simulink model "SIXDOF28"  (R2025b)
settings: Solver=VariableStepAuto  StartTime=0.0  StopTime=sortieStopTime_s  MaxStep=2.0  RelTol=1e-3
undefined symbols (not defined in the file): aircraft_mass, alpha0, alpha_bp, b, CL_table, ClCsurfaces, Cldampingrates, Cldeltae, CmCsurfaces, Cmdampingrates, CnCsurfaces, Cndampingrates, COP, CruiseSpeed, deg, density, DiscIntNeverNeededParam, dwGrad, ElTrim, g, h0, InitialHeadingRadBySortie, InitialPosBySortie, InitPitch, InitUb, Initwb, l, lt, maxPropRad, payloadvolume, PitchTrim, rad, rho, s, S, selectedSortie, St, ThrottleTrim
libraries: slpidlib x12, aerolibasang x3, aerolibconvert2 x2, aerolibadyn x1
(part 1 of 3)
settings Model: Creator=User  LastModifiedBy=User
settings SolverCC: ZeroCrossAlgorithm=Adaptive
settings DataIOCC: ExternalInput=getinputstruct(SIXDOF17TRIM)  InitialState=getstatestruct(SIXDOF17TRIM)  Refine=5
settings DebuggingCC: MaskedZcDiagnostic=none  IgnoredZcDiagnostic=none

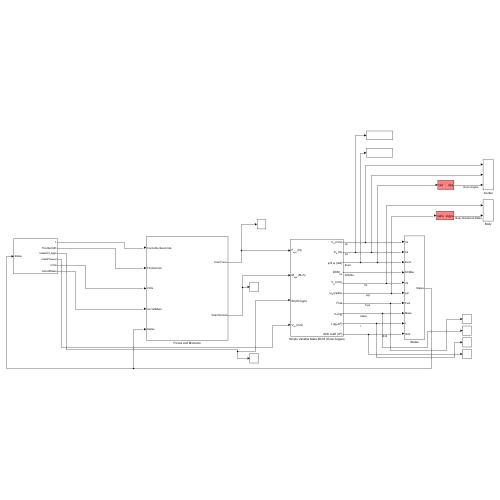
[thumbnail: Simulink's stored preview of the top-level diagram]
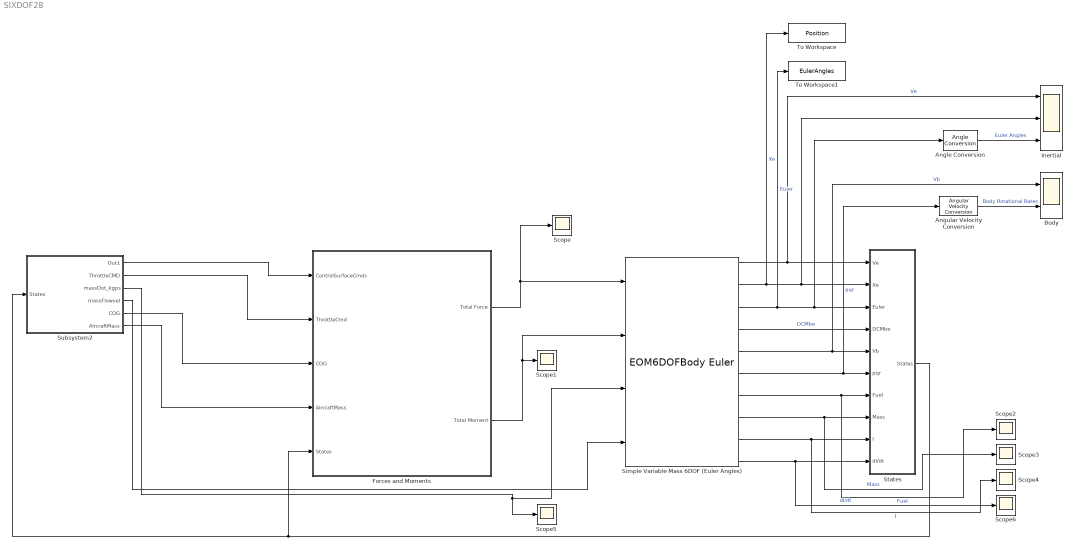
== system SIXDOF28 ==
  Angle Conversion : aerolibconvert2/Angle Conversion  IU=rad  OU=deg
  Angular Velocity Conversion : aerolibconvert2/Angular Velocity Conversion  IU=rad/s  OU=deg/s
  Body : Scope  NumInputPorts=2
      settings: TimeSpan=10  ActiveDisplayYMinimum=-7.1173373143171261  ActiveDisplayYMaximum=39.342522904173691
  Forces and Moments : Subsystem
  Inertial : Scope  NumInputPorts=3
      settings: TimeSpan=10  ActiveDisplayYMinimum=-30.17741938857975  ActiveDisplayYMaximum=31.493242322208388  DataLoggingVariableName=InertialData
  Scope{,1..6} (7 alike) : Scope
      Scope settings: ActiveDisplayYMinimum=-1086.3345140909432  ActiveDisplayYMaximum=956.25135632506715  DataLoggingVariableName=ScopeData65
      Scope1 settings: ActiveDisplayYMinimum=-0.001966592183015876  ActiveDisplayYMaximum=0.0097082532484662285  DataLoggingVariableName=ScopeData66
      Scope2 settings: ActiveDisplayYMinimum=-1  ActiveDisplayYMaximum=1  DataLoggingVariableName=ScopeData57
      Scope3 settings: ActiveDisplayYMinimum=92.2325499999995  ActiveDisplayYMaximum=150.86305000000004  DataLoggingVariableName=ScopeData60
      Scope4 settings: DataLoggingVariableName=ScopeData82
      Scope5 settings: ActiveDisplayYMinimum=-1  ActiveDisplayYMaximum=1  DataLoggingVariableName=ScopeData120
      Scope6 settings: DataLoggingVariableName=ScopeData92
  Simple Variable Mass 6DOF (Euler Angles) : EOM6DOFBodyEuler  mtype=Simple Variable  xme_0=InitialPosBySortie(selectedSortie,:)  Vm_0=[InitUb 0 Initwb]  eul_0=[0 InitPitch InitialHeadingRadBySortie(selectedSortie)]  mass_0=aircraft_mass  mass_e=emptymass  mass_f=aircraft_mass  inertia_e=EmptyInertiaMatrix  inertia_f=FullInertiaMatrix  vre_flag=on  mass_flag=on
  States : Subsystem
  Subsystem2 : Subsystem
  To Workspace : ToWorkspace  VariableName=Position  SaveFormat=Timeseries  SampleTime=-1
  To Workspace1 : ToWorkspace  VariableName=EulerAngles  SaveFormat=Timeseries  SampleTime=-1
  wires:
  Angle Conversion/1 -> Inertial/3  "Euler Angles"
  Angular Velocity Conversion/1 -> Body/2  "Body Rotational Rates"
  States/1(States) -> Subsystem2/1(States), Forces and Moments/5(States)
  Subsystem2/1(Out1) -> Forces and Moments/1(ControlSurfaceCmds)
  Forces and Moments/1(Total Force) -> Simple Variable Mass 6DOF (Euler Angles)/1, Scope/1
  Forces and Moments/2(Total Moment) -> Simple Variable Mass 6DOF (Euler Angles)/2, Scope1/1
  Subsystem2/2(ThrottleCMD) -> Forces and Moments/2(ThrottleCmd)
  Subsystem2/3(massDot_kgps) -> Simple Variable Mass 6DOF (Euler Angles)/3, Scope5/1
  Subsystem2/4(massFlowvel) -> Simple Variable Mass 6DOF (Euler Angles)/4
  Subsystem2/5(COG) -> Forces and Moments/3(COG)
  Subsystem2/6(AircraftMass) -> Forces and Moments/4(AircraftMass)
  Simple Variable Mass 6DOF (Euler Angles)/1 -> States/1(Ve), Inertial/1  "Ve"
  Simple Variable Mass 6DOF (Euler Angles)/2 -> To Workspace/1, States/2(Xe), Inertial/2  "Xe"
  Simple Variable Mass 6DOF (Euler Angles)/3 -> To Workspace1/1, States/3(Euler), Angle Conversion/1  "Euler"
  Simple Variable Mass 6DOF (Euler Angles)/4 -> States/4(DCMbe)  "DCMbe"
  Simple Variable Mass 6DOF (Euler Angles)/5 -> Body/1, States/5(Vb)  "Vb"
  Simple Variable Mass 6DOF (Euler Angles)/6 -> Angular Velocity Conversion/1, States/6(pqr)  "pqr"
  Simple Variable Mass 6DOF (Euler Angles)/7 -> Scope2/1, States/7(Fuel)  "Fuel"
  Simple Variable Mass 6DOF (Euler Angles)/8 -> Scope3/1, States/8(Mass)  "Mass"
  Simple Variable Mass 6DOF (Euler Angles)/9 -> Scope4/1, States/9(I)  "I"
  Simple Variable Mass 6DOF (Euler Angles)/10 -> Scope6/1, States/10(dI/dt)  "dI/dt"

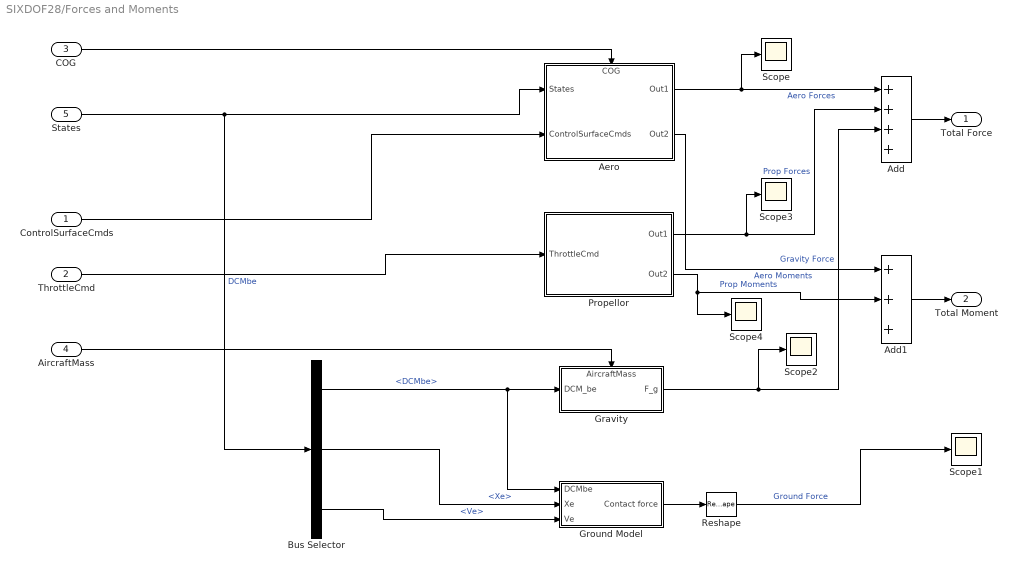
== system SIXDOF28/Forces and Moments ==
  ControlSurfaceCmds : Inport
  ThrottleCmd : Inport  Port=2
  COG : Inport  Port=3
  AircraftMass : Inport  Port=4
  States : Inport  Port=5
  Add : Sum  Inputs=++++
  Add1 : Sum  Inputs=+++
  Aero : Subsystem
      settings: PortSchema="{\"entries\":[{\"content\":{\"sides\":[{\"content\":{\"connectorIds\":[\"In1\",\"In2\"]},\"type\":\"ConnectorPlacement.EquallySpacedRectSide\",\"uuid\":\"609f64a6-fe2d-463f-8571-6107a2609829\"},{\"content\":{\"connectorIds\":[\"Out1\",\"Out2\"],\"side\":\"RIGHT\"},\"type\":\"ConnectorPlacement.EquallySpacedRectSide\",\"uuid\":\"636f2898-b73d-43f5-aead-2dc1a8211e6d\"},{\"content\":{\"connectorIds\":[\"In3\"],\"side\":\"TOP\"},\"type\":\"ConnectorPlacement.EquallySpacedRectSide\",\"uuid\":\"2beb2726-5e66-44a5-8496-281bf40e3bd0\"}]},\"type\":\"ConnectorPlacement.EquallySpacedConnector\",\"uuid\":\"f99eef0b-ac9c-4788-9a1a-1fc150c0b76e\"}],\"packageUris\":[\"http://schema.mathworks.com/mf0/Connector/R2020b\"],\"version\":\"1.0\"}"
  Bus Selector : BusSelector  OutputSignals=DCMbe,Xe,Ve
  Gravity : Subsystem
      settings: PortSchema="{\"entries\":[{\"content\":{\"sides\":[{\"content\":{\"connectorIds\":[\"In1\"]},\"type\":\"ConnectorPlacement.EquallySpacedRectSide\",\"uuid\":\"63d9ec0b-6663-4eeb-9ffd-c4a1f3d6fae8\"},{\"content\":{\"connectorIds\":[\"Out1\"],\"side\":\"RIGHT\"},\"type\":\"ConnectorPlacement.EquallySpacedRectSide\",\"uuid\":\"9033ce56-a827-4af9-9d8f-92169c025264\"},{\"content\":{\"connectorIds\":[\"In2\"],\"side\":\"TOP\"},\"type\":\"ConnectorPlacement.EquallySpacedRectSide\",\"uuid\":\"84568abc-cdbf-45a7-a6af-9a5fdbdb6515\"}]},\"type\":\"ConnectorPlacement.EquallySpacedConnector\",\"uuid\":\"857b6717-75e8-42d2-8d9f-18d4eadb3b26\"}],\"packageUris\":[\"http://schema.mathworks.com/mf0/Connector/R2020b\"],\"version\":\"1.0\"}"
  Ground Model : Subsystem
  Propellor : Subsystem
  Reshape : Reshape
  Scope{,1..4} (5 alike) : Scope
      Scope settings: ActiveDisplayYMinimum=-2618.1799390430056  ActiveDisplayYMaximum=542.63664124652109  DataLoggingVariableName=ScopeData40
      Scope1 settings: ActiveDisplayYMinimum=-1  ActiveDisplayYMaximum=1  DataLoggingVariableName=ScopeData43
      Scope2 settings: ActiveDisplayYMinimum=-236.10201419942058  ActiveDisplayYMaximum=1116.233557133269  DataLoggingVariableName=ScopeData44
      Scope3 settings: ActiveDisplayYMinimum=-38.137986036605241  ActiveDisplayYMaximum=343.24187432944723  DataLoggingVariableName=ScopeData54
      Scope4 settings: ActiveDisplayYMinimum=-19.196026162968661  ActiveDisplayYMaximum=172.764235466718  DataLoggingVariableName=ScopeData80
  Total Force : Outport
  Total Moment : Outport  Port=2
  wires:
  Add/1 -> Total Force/1
  Add1/1 -> Total Moment/1
  States/1 -> Bus Selector/1, Aero/1(States)  "DCMbe"
  Bus Selector/1 -> Ground Model/1(DCMbe), Gravity/1(DCM_be)  "<DCMbe>"
  Bus Selector/2 -> Ground Model/2(Xe)  "<Xe>"
  Bus Selector/3 -> Ground Model/3(Ve)  "<Ve>"
  Ground Model/1(Contact force) -> Reshape/1
  Reshape/1 -> Scope1/1  "Ground Force"
  Aero/1(Out1) -> Add/1, Scope/1  "Aero Forces"
  Gravity/1(F_g) -> Scope2/1, Add/3  "Gravity Force"
  ControlSurfaceCmds/1 -> Aero/2(ControlSurfaceCmds)
  Propellor/1(Out1) -> Scope3/1, Add/2  "Prop Forces"
  ThrottleCmd/1 -> Propellor/1(ThrottleCmd)
  Propellor/2(Out2) -> Add1/2, Scope4/1  "Prop Moments"
  Aero/2(Out2) -> Add1/1  "Aero Moments"
  COG/1 -> Aero/3(COG)
  AircraftMass/1 -> Gravity/2(AircraftMass)

== system SIXDOF28/States ==
  Ve : Inport
  Xe : Inport  Port=2
  Euler : Inport  Port=3
  DCMbe : Inport  Port=4
  Vb : Inport  Port=5
  pqr : Inport  Port=6
  Fuel : Inport  Port=7
  Mass : Inport  Port=8
  I : Inport  Port=9
  dI/dt : Inport  Port=10
  Atan2 : Trigonometry  Operator=atan2
  Bus Creator : BusCreator  Inputs=11
  Selector : Selector  InputPortWidth=3  IndexOptions=Index vector (dialog)  Indices=[2]  OutputSizes=1
  Selector1 : Selector  InputPortWidth=3  IndexOptions=Index vector (dialog)  Indices=[1]  OutputSizes=1
  States : Outport
  wires:
  Bus Creator/1 -> States/1
  Ve/1 -> Selector1/1, Selector/1, Bus Creator/1
  Xe/1 -> Bus Creator/2
  Euler/1 -> Bus Creator/3
  DCMbe/1 -> Bus Creator/4
  Vb/1 -> Bus Creator/5
  pqr/1 -> Bus Creator/6
  Fuel/1 -> Bus Creator/7
  Mass/1 -> Bus Creator/8
  I/1 -> Bus Creator/9
  Selector/1 -> Atan2/1
  Selector1/1 -> Atan2/2
  Atan2/1 -> Bus Creator/11  "Heading"
  dI/dt/1 -> Bus Creator/10

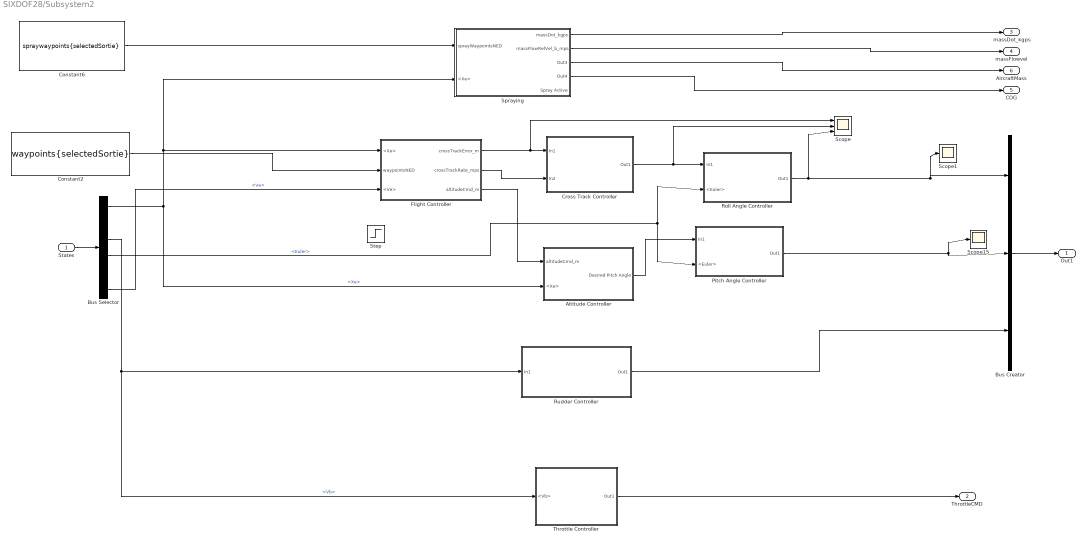
== system SIXDOF28/Subsystem2 ==
  States : Inport
  Altitude Controller : Subsystem
  Bus Creator : BusCreator  Inputs=3
  Bus Selector : BusSelector  OutputSignals=Xe,pqr,Vb,Euler,Heading,Ve
  Constant2 : Constant  Value=waypoints{selectedSortie}
  Constant6 : Constant  Value=spraywaypoints{selectedSortie}
  Cross Track Controller : Subsystem
  Flight Controller : Subsystem
  Pitch Angle Controller : Subsystem
  Roll Angle Controller : Subsystem
  Rudder Controller : Subsystem
  Scope : Scope  NumInputPorts=3
      settings: ActiveDisplayYMinimum=-1  ActiveDisplayYMaximum=1  DataLoggingVariableName=ScopeData85
  Scope1 : Scope
      settings: DataLoggingVariableName=ScopeData86
  Scope15 : Scope
      settings: ActiveDisplayYMinimum=-0.51269046777333427  ActiveDisplayYMaximum=0.25089107997418486  DataLoggingVariableName=ScopeData84
  Spraying : Subsystem
  Step : Step  Time=50  Before=4  After=20  SampleTime=0
  Throttle Controller : Subsystem
  Out1 : Outport
  ThrottleCMD : Outport  Port=2
  massDot_kgps : Outport  Port=3
  massFlowvel : Outport  Port=4
  COG : Outport  Port=5
  AircraftMass : Outport  Port=6
  wires:
  States/1 -> Bus Selector/1
  Bus Creator/1 -> Out1/1
  Altitude Controller/1(Desired Pitch Angle) -> Pitch Angle Controller/1(In1)
  Bus Selector/1 -> Altitude Controller/2(<Xe>), Spraying/2(<Xe>), Flight Controller/1(<Xe>)  "<Xe>"
  Pitch Angle Controller/1(Out1) -> Bus Creator/2, Scope15/1
  Bus Selector/4 -> Pitch Angle Controller/2(<Euler>), Roll Angle Controller/2(<Euler>)  "<Euler>"
  Roll Angle Controller/1(Out1) -> Scope/3, Bus Creator/1, Scope1/1
  Bus Selector/3 -> Rudder Controller/1(In1), Throttle Controller/1(<Vb>)  "<Vb>"
  Throttle Controller/1(Out1) -> ThrottleCMD/1
  Cross Track Controller/1(Out1) -> Scope/2, Roll Angle Controller/1(In1)
  Bus Selector/6 -> Flight Controller/3(<Ve>)  "<Ve>"
  Flight Controller/1(crossTrackError_m) -> Scope/1, Cross Track Controller/1(In1)
  Flight Controller/2(crossTrackRate_mps) -> Cross Track Controller/2(In2)
  Spraying/1(massDot_kgps) -> massDot_kgps/1
  Spraying/2(massFlowRelVel_b_mps) -> massFlowvel/1
  Spraying/3(Out3) -> AircraftMass/1
  Spraying/4(Out4) -> COG/1
  Flight Controller/3(altitudeCmd_m) -> Altitude Controller/1(altitudeCmd_m)
  Constant2/1 -> Flight Controller/2(waypointsNED)
  Constant6/1 -> Spraying/1(sprayWaypointsNED)
  Rudder Controller/1(Out1) -> Bus Creator/3

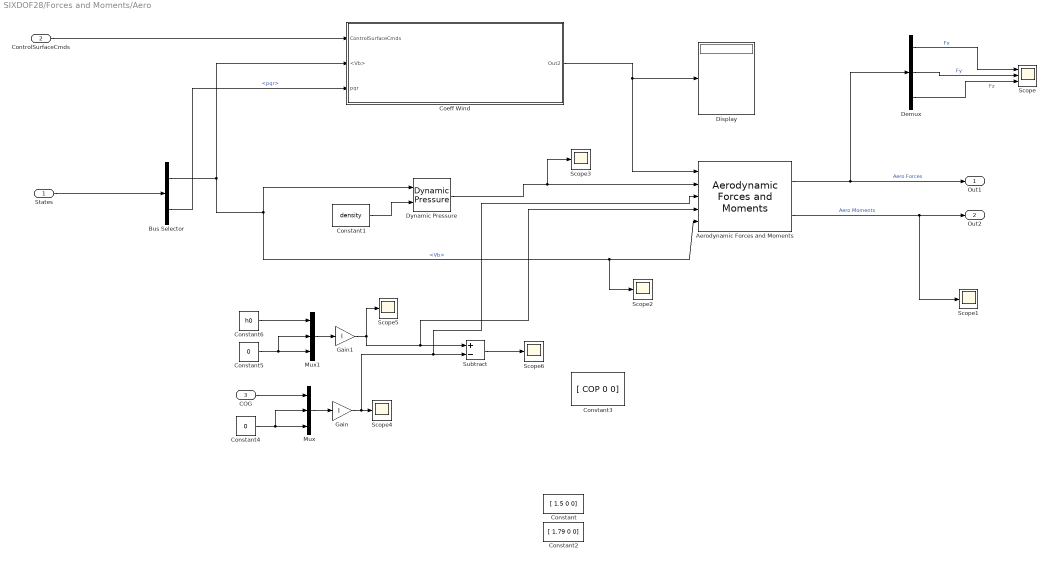
== system SIXDOF28/Forces and Moments/Aero ==
  States : Inport
  ControlSurfaceCmds : Inport  Port=2
  COG : Inport  Port=3
  "Aerodynamic Forces and Moments " : aerolibadyn/Aerodynamic Forces and Moments   inputAxes=Wind  outputForceAxes=Body  outputMomentAxes=Body  S=S  b=b  cbar=l
  Bus Selector : BusSelector  OutputSignals=Vb,pqr
  Coeff Wind : Subsystem
  Constant : Constant  Value=[ 1.5 0 0]
  Constant1 : Constant  Value=density
  Constant2 : Constant  Value=[ 1.79 0 0]
  Constant3 : Constant  Value=[ COP 0 0]
  Constant4 : Constant  Value=0
  Constant5 : Constant  Value=0
  Constant6 : Constant  Value=h0
  Demux : Demux  Outputs=3
  Display : Display
  Dynamic Pressure : aerolibasang/Dynamic Pressure
  Gain : Gain  Gain=l
  Gain1 : Gain  Gain=l
  Mux : Mux  Inputs=3
  Mux1 : Mux  Inputs=3
  Scope : Scope  NumInputPorts=3
      settings: ActiveDisplayYMinimum=-2654.35797194935  ActiveDisplayYMaximum=770.34591129163266  DataLoggingVariableName=ScopeData13
  Scope{1..6} (6 alike) : Scope
      Scope1 settings: ActiveDisplayYMinimum=-1  ActiveDisplayYMaximum=1  DataLoggingVariableName=ScopeData14
      Scope2 settings: ActiveDisplayYMinimum=-1  ActiveDisplayYMaximum=1
      Scope3 settings: ActiveDisplayYMinimum=-1  ActiveDisplayYMaximum=1  DataLoggingVariableName=ScopeData2
      Scope4 settings: ActiveDisplayYMinimum=-1  ActiveDisplayYMaximum=1  DataLoggingVariableName=ScopeData125
      Scope5 settings: ActiveDisplayYMinimum=-1  ActiveDisplayYMaximum=1  DataLoggingVariableName=ScopeData126
      Scope6 settings: ActiveDisplayYMinimum=-1  ActiveDisplayYMaximum=1  DataLoggingVariableName=ScopeData127
  Subtract : Sum  Inputs=+-
  Out1 : Outport
  Out2 : Outport  Port=2
  wires:
  "Aerodynamic Forces and Moments "/1 -> Demux/1, Out1/1  "Aero Forces"
  "Aerodynamic Forces and Moments "/2 -> Scope1/1, Out2/1  "Aero Moments"
  Constant1/1 -> Dynamic Pressure/2
  Dynamic Pressure/1 -> Scope3/1, "Aerodynamic Forces and Moments "/2
  States/1 -> Bus Selector/1
  Bus Selector/1 -> Scope2/1, "Aerodynamic Forces and Moments "/5, Dynamic Pressure/1, Coeff Wind/2(<Vb>)  "<Vb>"
  Coeff Wind/1(Out2) -> "Aerodynamic Forces and Moments "/1, Display/1
  Demux/2 -> Scope/2  "Fy"
  Demux/1 -> Scope/1  "Fx"
  Demux/3 -> Scope/3  "Fz"
  Bus Selector/2 -> Coeff Wind/3(pqr)  "<pqr>"
  ControlSurfaceCmds/1 -> Coeff Wind/1(ControlSurfaceCmds)
  COG/1 -> Mux/1
  Constant4/1 -> Mux/2, Mux/3
  Mux/1 -> Gain/1
  Gain/1 -> "Aerodynamic Forces and Moments "/3, Subtract/2, Scope4/1
  Constant5/1 -> Mux1/2, Mux1/3
  Constant6/1 -> Mux1/1
  Mux1/1 -> Gain1/1
  Gain1/1 -> Scope5/1, "Aerodynamic Forces and Moments "/4, Subtract/1
  Subtract/1 -> Scope6/1

== system SIXDOF28/Forces and Moments/Gravity ==
  DCM_be : Inport
  AircraftMass : Inport  Port=2
  Constant : Constant  Value=[ 0 0 g]
  MatrixMultiply : Product  Multiplication=Matrix(*)
  Product : Product
  F_g : Outport
  wires:
  Constant/1 -> MatrixMultiply/2
  DCM_be/1 -> MatrixMultiply/1
  MatrixMultiply/1 -> Product/2
  Product/1 -> F_g/1
  AircraftMass/1 -> Product/1

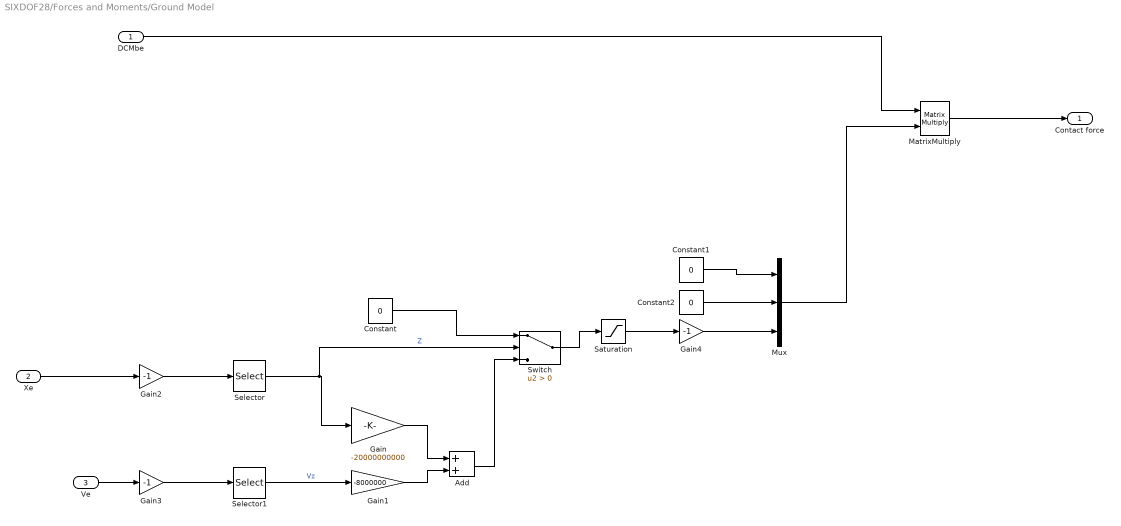
== system SIXDOF28/Forces and Moments/Ground Model ==
  DCMbe : Inport
  Xe : Inport  Port=2
  Ve : Inport  Port=3
  Add : Sum
  Constant : Constant  Value=0
  Constant1 : Constant  Value=0
  Constant2 : Constant  Value=0
  Gain : Gain  Gain=-20000000000
  Gain1 : Gain  Gain=-8000000
  Gain2 : Gain  Gain=-1
  Gain3 : Gain  Gain=-1
  Gain4 : Gain  Gain=-1
  MatrixMultiply : Product  Multiplication=Matrix(*)
  Mux : Mux  Inputs=3
  Saturation : Saturate  UpperLimit=inf  LowerLimit=-0.0
  Selector : Selector  InputPortWidth=3  IndexOptions=Index vector (dialog)  Indices=[3]  OutputSizes=1
  Selector1 : Selector  InputPortWidth=3  IndexOptions=Index vector (dialog)  Indices=[3]  OutputSizes=1
  Switch : Switch  Criteria=u2 > Threshold  SaturateOnIntegerOverflow=off  InputSameDT=off
  Contact force : Outport
  wires:
  Xe/1 -> Gain2/1
  Ve/1 -> Gain3/1
  Constant/1 -> Switch/1
  Gain/1 -> Add/1
  Gain1/1 -> Add/2
  Selector1/1 -> Gain1/1  "Vz"
  Selector/1 -> Switch/2, Gain/1  "Z"
  Add/1 -> Switch/3
  Gain2/1 -> Selector/1
  Gain3/1 -> Selector1/1
  Switch/1 -> Saturation/1
  DCMbe/1 -> MatrixMultiply/1
  MatrixMultiply/1 -> Contact force/1
  Gain4/1 -> Mux/3
  Constant2/1 -> Mux/2
  Constant1/1 -> Mux/1
  Saturation/1 -> Gain4/1
  Mux/1 -> MatrixMultiply/2

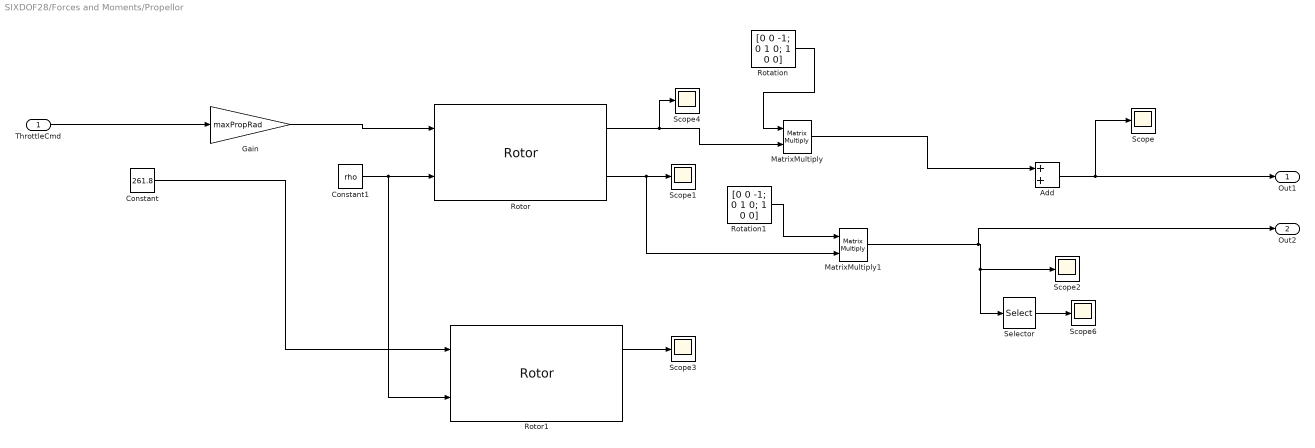
== system SIXDOF28/Forces and Moments/Propellor ==
  ThrottleCmd : Inport
  Add : Sum
  Constant : Constant  Value=261.8
  Constant1 : Constant  Value=rho
  Gain : Gain  Gain=maxPropRad
  MatrixMultiply : Product  Multiplication=Matrix(*)
  MatrixMultiply1 : Product  Multiplication=Matrix(*)
  Rotation : Constant  Value=[0 0 -1; 0 1 0; 1 0 0]
  Rotation1 : Constant  Value=[0 0 -1; 0 1 0; 1 0 0]
  Rotor : Rotor  CT=CT  CQ=CQ  radius=PropRadius
  Rotor1 : Rotor  radius=PropRadius
  Scope{,1..4,6} (6 alike) : Scope
      Scope settings: ActiveDisplayYMinimum=-1  ActiveDisplayYMaximum=1  DataLoggingVariableName=ScopeData18
      Scope1 settings: ActiveDisplayYMinimum=-1  ActiveDisplayYMaximum=1  DataLoggingVariableName=ScopeData19
      Scope2 settings: ActiveDisplayYMinimum=-0.90688934039232  ActiveDisplayYMaximum=8.1620040635308833  DataLoggingVariableName=ScopeData71
      Scope3 settings: ActiveDisplayYMinimum=-1  ActiveDisplayYMaximum=1  DataLoggingVariableName=ScopeData52
      Scope4 settings: ActiveDisplayYMinimum=-1  ActiveDisplayYMaximum=1  DataLoggingVariableName=ScopeData72
      Scope6 settings: ActiveDisplayYMinimum=-1  ActiveDisplayYMaximum=1  DataLoggingVariableName=ScopeData73
  Selector : Selector  InputPortWidth=3  IndexOptions=Index vector (dialog)  Indices=[ 1]  OutputSizes=1
  Out1 : Outport
  Out2 : Outport  Port=2
  wires:
  Constant1/1 -> Rotor1/2, Rotor/2
  Rotor/2 -> MatrixMultiply1/2, Scope1/1
  Add/1 -> Scope/1, Out1/1
  Rotor/1 -> Scope4/1, MatrixMultiply/2
  Rotation/1 -> MatrixMultiply/1
  MatrixMultiply/1 -> Add/1
  ThrottleCmd/1 -> Gain/1
  Rotation1/1 -> MatrixMultiply1/1
  MatrixMultiply1/1 -> Out2/1, Selector/1, Scope2/1
  Selector/1 -> Scope6/1
  Constant/1 -> Rotor1/1
  Rotor1/1 -> Scope3/1
  Gain/1 -> Rotor/1

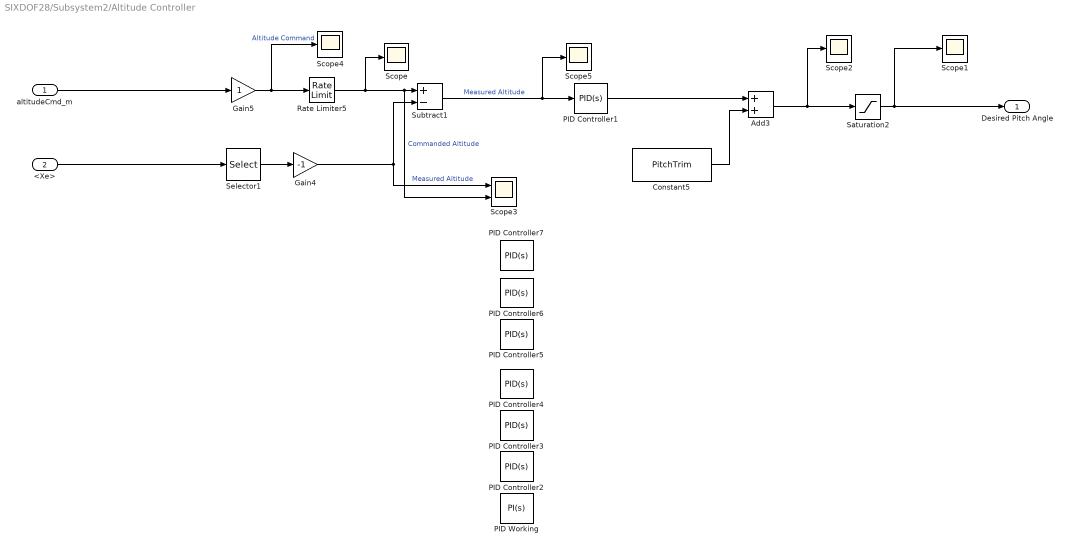
== system SIXDOF28/Subsystem2/Altitude Controller ==
  altitudeCmd_m : Inport
  <Xe> : Inport  Port=2
  Add3 : Sum
  Constant5 : Constant  Value=PitchTrim
  Gain4 : Gain  Gain=-1
  Gain5 : Gain
  PID Controller1 : slpidlib/PID Controller  Controller=PID  Form=Parallel  TimeDomain=Continuous-time  UseExternalTs=off  SampleTime=-1  IntegratorMethod=Forward Euler  FilterMethod=Forward Euler  ControllerParametersSource=internal  P=0.095  I=0.01  UseKiTs=off  D=0.07  UseExternalDerivativeSource=off  N=100  UseFilter=on  TunerSelectOption=Transfer Function Based (PID Tuner App)  InitialConditionSource=internal  InitialConditionForIntegrator=0  InitialConditionForFilter=0  DifferentiatorICPrevScaledInput=0  ExternalReset=none  TrackingMode=off  Kt=1  LimitOutput=off  SatLimitsSource=internal  UpperSaturationLimit=inf  LowerSaturationLimit=-inf  LinearizeAsGain=on  AntiWindupMode=none  Kb=1  LimitIntegrator=off  UpperIntegratorSaturationLimit=inf  LowerIntegratorSaturationLimit=-inf  POutMin=[]  POutMax=[]  IOutMin=[]  IOutMax=[]  DOutMin=[]  DOutMax=[]  NOutMin=[]  NOutMax=[]  SumOutMin=[]  SumOutMax=[]  SaturationOutMin=[]  SaturationOutMax=[]  PParamMin=[]  PParamMax=[]  IParamMin=[]  IParamMax=[]  DParamMin=[]  DParamMax=[]  NParamMin=[]  NParamMax=[]  KbParamMin=[]  KbParamMax=[]  KtParamMin=[]  KtParamMax=[]  KbOutMin=[]  KbOutMax=[]  KtOutMin=[]  KtOutMax=[]  IntegratorOutMin=[]  IntegratorOutMax=[]  FilterOutMin=[]  FilterOutMax=[]  SumI1OutMin=[]  SumI1OutMax=[]  SumI2OutMin=[]  SumI2OutMax=[]  SumI3OutMin=[]  SumI3OutMax=[]  SumI4OutMin=[]  SumI4OutMax=[]  SumDOutMin=[]  SumDOutMax=[]  DifferentiatorOutMin=[]  DifferentiatorOutMax=[]  FilterDiffOutCoefMin=[]  FilterDiffOutCoefMax=[]  ReciprocalOutMin=[]  ReciprocalOutMax=[]  SumDenOutMin=[]  SumDenOutMax=[]  SumNumOutMin=[]  SumNumOutMax=[]  DivideOutMin=[]  DivideOutMax=[]  UdiffTsProdOutMin=[]  UdiffTsProdOutMax=[]  NTsProdOutMin=[]  NTsProdOutMax=[]  UintegralTsProdOutMin=[]  UintegralTsProdOutMax=[]  UngainTsProdOutMin=[]  UngainTsProdOutMax=[]  ClampingZeroOutDataTypeStr=Inherit: Inherit via back propagation  ClampingZeroOutMin=[]  ClampingZeroOutMax=[]  FilterDenConstantOutDataTypeStr=Inherit: Inherit via back propagation  FilterDenConstantOutMin=[]  FilterDenConstantOutMax=[]  PCopyOutDataTypeStr=Inherit: Inherit via back propagation  PCopyOutMin=[]  PCopyOutMax=[]  NCopyOutDataTypeStr=Inherit: Inherit via back propagation  NCopyOutMin=[]  NCopyOutMax=[]  IntegratorContinuousStateAttributes=''  IntegratorStateMustResolveToSignalObject=off  IntegratorRTWStateStorageClass=Auto  FilterContinuousStateAttributes=''  FilterStateMustResolveToSignalObject=off  FilterRTWStateStorageClass=Auto  ParallelPVariant=InternalParameters  IdealPVariant=Disabled  IVariant=InternalParameters  DVariant=InternalParameters  IntegratorVariant=Continuous  SatVariant=Disabled  AWVariant=Passthrough  PCopyVariant=Disabled  TRVariant=Disabled  FdbkBlocksVariant=Forward  IdealPFdbkVariant=Disabled  SatFdbkVariant=Disabled  DerivativeFilterVariant=ContFilter  NVariant=InternalParameters  NCopyVariant=Disabled  FilterICVariant=InternalICsFilter  IntegratorICVariant=InternalICs  ExternalResetVariant=Disabled  TRSumVariant=Passthrough  SumFdbkVariant=Disabled  SumVariant=Sum_PID  TsampFilterVariant=InternalTs  TsampNgainVariant=Passthrough  TsampIntegralVariant=Disabled_SignalSpec  ExternalSaturationOutDataTypeStr=Inherit: Same as second input  DerivativeSourceVariant=ErrorSignal  PreIntVariant=InternalPreInt
  PID Controller2 : slpidlib/PID Controller  Controller=PID  Form=Parallel  TimeDomain=Continuous-time  UseExternalTs=off  SampleTime=-1  IntegratorMethod=Forward Euler  FilterMethod=Forward Euler  ControllerParametersSource=internal  P=0.1  I=0.01  UseKiTs=off  D=0.03  UseExternalDerivativeSource=off  N=100  UseFilter=on  TunerSelectOption=Transfer Function Based (PID Tuner App)  InitialConditionSource=internal  InitialConditionForIntegrator=0  InitialConditionForFilter=0  DifferentiatorICPrevScaledInput=0  ExternalReset=none  TrackingMode=off  Kt=1  LimitOutput=off  SatLimitsSource=internal  UpperSaturationLimit=inf  LowerSaturationLimit=-inf  LinearizeAsGain=on  AntiWindupMode=none  Kb=1  LimitIntegrator=off  UpperIntegratorSaturationLimit=inf  LowerIntegratorSaturationLimit=-inf  POutMin=[]  POutMax=[]  IOutMin=[]  IOutMax=[]  DOutMin=[]  DOutMax=[]  NOutMin=[]  NOutMax=[]  SumOutMin=[]  SumOutMax=[]  SaturationOutMin=[]  SaturationOutMax=[]  PParamMin=[]  PParamMax=[]  IParamMin=[]  IParamMax=[]  DParamMin=[]  DParamMax=[]  NParamMin=[]  NParamMax=[]  KbParamMin=[]  KbParamMax=[]  KtParamMin=[]  KtParamMax=[]  KbOutMin=[]  KbOutMax=[]  KtOutMin=[]  KtOutMax=[]  IntegratorOutMin=[]  IntegratorOutMax=[]  FilterOutMin=[]  FilterOutMax=[]  SumI1OutMin=[]  SumI1OutMax=[]  SumI2OutMin=[]  SumI2OutMax=[]  SumI3OutMin=[]  SumI3OutMax=[]  SumI4OutMin=[]  SumI4OutMax=[]  SumDOutMin=[]  SumDOutMax=[]  DifferentiatorOutMin=[]  DifferentiatorOutMax=[]  FilterDiffOutCoefMin=[]  FilterDiffOutCoefMax=[]  ReciprocalOutMin=[]  ReciprocalOutMax=[]  SumDenOutMin=[]  SumDenOutMax=[]  SumNumOutMin=[]  SumNumOutMax=[]  DivideOutMin=[]  DivideOutMax=[]  UdiffTsProdOutMin=[]  UdiffTsProdOutMax=[]  NTsProdOutMin=[]  NTsProdOutMax=[]  UintegralTsProdOutMin=[]  UintegralTsProdOutMax=[]  UngainTsProdOutMin=[]  UngainTsProdOutMax=[]  ClampingZeroOutDataTypeStr=Inherit: Inherit via back propagation  ClampingZeroOutMin=[]  ClampingZeroOutMax=[]  FilterDenConstantOutDataTypeStr=Inherit: Inherit via back propagation  FilterDenConstantOutMin=[]  FilterDenConstantOutMax=[]  PCopyOutDataTypeStr=Inherit: Inherit via back propagation  PCopyOutMin=[]  PCopyOutMax=[]  NCopyOutDataTypeStr=Inherit: Inherit via back propagation  NCopyOutMin=[]  NCopyOutMax=[]  IntegratorContinuousStateAttributes=''  IntegratorStateMustResolveToSignalObject=off  IntegratorRTWStateStorageClass=Auto  FilterContinuousStateAttributes=''  FilterStateMustResolveToSignalObject=off  FilterRTWStateStorageClass=Auto  ParallelPVariant=InternalParameters  IdealPVariant=Disabled  IVariant=InternalParameters  DVariant=InternalParameters  IntegratorVariant=Continuous  SatVariant=Disabled  AWVariant=Passthrough  PCopyVariant=Disabled  TRVariant=Disabled  FdbkBlocksVariant=Forward  IdealPFdbkVariant=Disabled  SatFdbkVariant=Disabled  DerivativeFilterVariant=ContFilter  NVariant=InternalParameters  NCopyVariant=Disabled  FilterICVariant=InternalICsFilter  IntegratorICVariant=InternalICs  ExternalResetVariant=Disabled  TRSumVariant=Passthrough  SumFdbkVariant=Disabled  SumVariant=Sum_PID  TsampFilterVariant=InternalTs  TsampNgainVariant=Passthrough  TsampIntegralVariant=Disabled_SignalSpec  ExternalSaturationOutDataTypeStr=Inherit: Same as second input  DerivativeSourceVariant=ErrorSignal  PreIntVariant=InternalPreInt
  PID Controller3 : slpidlib/PID Controller  Controller=PID  Form=Parallel  TimeDomain=Continuous-time  UseExternalTs=off  SampleTime=-1  IntegratorMethod=Forward Euler  FilterMethod=Forward Euler  ControllerParametersSource=internal  P=0.095  I=0.01  UseKiTs=off  D=0.03  UseExternalDerivativeSource=off  N=100  UseFilter=on  TunerSelectOption=Transfer Function Based (PID Tuner App)  InitialConditionSource=internal  InitialConditionForIntegrator=0  InitialConditionForFilter=0  DifferentiatorICPrevScaledInput=0  ExternalReset=none  TrackingMode=off  Kt=1  LimitOutput=off  SatLimitsSource=internal  UpperSaturationLimit=inf  LowerSaturationLimit=-inf  LinearizeAsGain=on  AntiWindupMode=none  Kb=1  LimitIntegrator=off  UpperIntegratorSaturationLimit=inf  LowerIntegratorSaturationLimit=-inf  POutMin=[]  POutMax=[]  IOutMin=[]  IOutMax=[]  DOutMin=[]  DOutMax=[]  NOutMin=[]  NOutMax=[]  SumOutMin=[]  SumOutMax=[]  SaturationOutMin=[]  SaturationOutMax=[]  PParamMin=[]  PParamMax=[]  IParamMin=[]  IParamMax=[]  DParamMin=[]  DParamMax=[]  NParamMin=[]  NParamMax=[]  KbParamMin=[]  KbParamMax=[]  KtParamMin=[]  KtParamMax=[]  KbOutMin=[]  KbOutMax=[]  KtOutMin=[]  KtOutMax=[]  IntegratorOutMin=[]  IntegratorOutMax=[]  FilterOutMin=[]  FilterOutMax=[]  SumI1OutMin=[]  SumI1OutMax=[]  SumI2OutMin=[]  SumI2OutMax=[]  SumI3OutMin=[]  SumI3OutMax=[]  SumI4OutMin=[]  SumI4OutMax=[]  SumDOutMin=[]  SumDOutMax=[]  DifferentiatorOutMin=[]  DifferentiatorOutMax=[]  FilterDiffOutCoefMin=[]  FilterDiffOutCoefMax=[]  ReciprocalOutMin=[]  ReciprocalOutMax=[]  SumDenOutMin=[]  SumDenOutMax=[]  SumNumOutMin=[]  SumNumOutMax=[]  DivideOutMin=[]  DivideOutMax=[]  UdiffTsProdOutMin=[]  UdiffTsProdOutMax=[]  NTsProdOutMin=[]  NTsProdOutMax=[]  UintegralTsProdOutMin=[]  UintegralTsProdOutMax=[]  UngainTsProdOutMin=[]  UngainTsProdOutMax=[]  ClampingZeroOutDataTypeStr=Inherit: Inherit via back propagation  ClampingZeroOutMin=[]  ClampingZeroOutMax=[]  FilterDenConstantOutDataTypeStr=Inherit: Inherit via back propagation  FilterDenConstantOutMin=[]  FilterDenConstantOutMax=[]  PCopyOutDataTypeStr=Inherit: Inherit via back propagation  PCopyOutMin=[]  PCopyOutMax=[]  NCopyOutDataTypeStr=Inherit: Inherit via back propagation  NCopyOutMin=[]  NCopyOutMax=[]  IntegratorContinuousStateAttributes=''  IntegratorStateMustResolveToSignalObject=off  IntegratorRTWStateStorageClass=Auto  FilterContinuousStateAttributes=''  FilterStateMustResolveToSignalObject=off  FilterRTWStateStorageClass=Auto  ParallelPVariant=InternalParameters  IdealPVariant=Disabled  IVariant=InternalParameters  DVariant=InternalParameters  IntegratorVariant=Continuous  SatVariant=Disabled  AWVariant=Passthrough  PCopyVariant=Disabled  TRVariant=Disabled  FdbkBlocksVariant=Forward  IdealPFdbkVariant=Disabled  SatFdbkVariant=Disabled  DerivativeFilterVariant=ContFilter  NVariant=InternalParameters  NCopyVariant=Disabled  FilterICVariant=InternalICsFilter  IntegratorICVariant=InternalICs  ExternalResetVariant=Disabled  TRSumVariant=Passthrough  SumFdbkVariant=Disabled  SumVariant=Sum_PID  TsampFilterVariant=InternalTs  TsampNgainVariant=Passthrough  TsampIntegralVariant=Disabled_SignalSpec  ExternalSaturationOutDataTypeStr=Inherit: Same as second input  DerivativeSourceVariant=ErrorSignal  PreIntVariant=InternalPreInt
  PID Controller4 : slpidlib/PID Controller  Controller=PID  Form=Parallel  TimeDomain=Continuous-time  UseExternalTs=off  SampleTime=-1  IntegratorMethod=Forward Euler  FilterMethod=Forward Euler  ControllerParametersSource=internal  P=0.1  I=0.01  UseKiTs=off  D=0.045  UseExternalDerivativeSource=off  N=100  UseFilter=on  TunerSelectOption=Transfer Function Based (PID Tuner App)  InitialConditionSource=internal  InitialConditionForIntegrator=0  InitialConditionForFilter=0  DifferentiatorICPrevScaledInput=0  ExternalReset=none  TrackingMode=off  Kt=1  LimitOutput=off  SatLimitsSource=internal  UpperSaturationLimit=inf  LowerSaturationLimit=-inf  LinearizeAsGain=on  AntiWindupMode=none  Kb=1  LimitIntegrator=off  UpperIntegratorSaturationLimit=inf  LowerIntegratorSaturationLimit=-inf  POutMin=[]  POutMax=[]  IOutMin=[]  IOutMax=[]  DOutMin=[]  DOutMax=[]  NOutMin=[]  NOutMax=[]  SumOutMin=[]  SumOutMax=[]  SaturationOutMin=[]  SaturationOutMax=[]  PParamMin=[]  PParamMax=[]  IParamMin=[]  IParamMax=[]  DParamMin=[]  DParamMax=[]  NParamMin=[]  NParamMax=[]  KbParamMin=[]  KbParamMax=[]  KtParamMin=[]  KtParamMax=[]  KbOutMin=[]  KbOutMax=[]  KtOutMin=[]  KtOutMax=[]  IntegratorOutMin=[]  IntegratorOutMax=[]  FilterOutMin=[]  FilterOutMax=[]  SumI1OutMin=[]  SumI1OutMax=[]  SumI2OutMin=[]  SumI2OutMax=[]  SumI3OutMin=[]  SumI3OutMax=[]  SumI4OutMin=[]  SumI4OutMax=[]  SumDOutMin=[]  SumDOutMax=[]  DifferentiatorOutMin=[]  DifferentiatorOutMax=[]  FilterDiffOutCoefMin=[]  FilterDiffOutCoefMax=[]  ReciprocalOutMin=[]  ReciprocalOutMax=[]  SumDenOutMin=[]  SumDenOutMax=[]  SumNumOutMin=[]  SumNumOutMax=[]  DivideOutMin=[]  DivideOutMax=[]  UdiffTsProdOutMin=[]  UdiffTsProdOutMax=[]  NTsProdOutMin=[]  NTsProdOutMax=[]  UintegralTsProdOutMin=[]  UintegralTsProdOutMax=[]  UngainTsProdOutMin=[]  UngainTsProdOutMax=[]  ClampingZeroOutDataTypeStr=Inherit: Inherit via back propagation  ClampingZeroOutMin=[]  ClampingZeroOutMax=[]  FilterDenConstantOutDataTypeStr=Inherit: Inherit via back propagation  FilterDenConstantOutMin=[]  FilterDenConstantOutMax=[]  PCopyOutDataTypeStr=Inherit: Inherit via back propagation  PCopyOutMin=[]  PCopyOutMax=[]  NCopyOutDataTypeStr=Inherit: Inherit via back propagation  NCopyOutMin=[]  NCopyOutMax=[]  IntegratorContinuousStateAttributes=''  IntegratorStateMustResolveToSignalObject=off  IntegratorRTWStateStorageClass=Auto  FilterContinuousStateAttributes=''  FilterStateMustResolveToSignalObject=off  FilterRTWStateStorageClass=Auto  ParallelPVariant=InternalParameters  IdealPVariant=Disabled  IVariant=InternalParameters  DVariant=InternalParameters  IntegratorVariant=Continuous  SatVariant=Disabled  AWVariant=Passthrough  PCopyVariant=Disabled  TRVariant=Disabled  FdbkBlocksVariant=Forward  IdealPFdbkVariant=Disabled  SatFdbkVariant=Disabled  DerivativeFilterVariant=ContFilter  NVariant=InternalParameters  NCopyVariant=Disabled  FilterICVariant=InternalICsFilter  IntegratorICVariant=InternalICs  ExternalResetVariant=Disabled  TRSumVariant=Passthrough  SumFdbkVariant=Disabled  SumVariant=Sum_PID  TsampFilterVariant=InternalTs  TsampNgainVariant=Passthrough  TsampIntegralVariant=Disabled_SignalSpec  ExternalSaturationOutDataTypeStr=Inherit: Same as second input  DerivativeSourceVariant=ErrorSignal  PreIntVariant=InternalPreInt
  PID Controller5 : slpidlib/PID Controller  Controller=PID  Form=Parallel  TimeDomain=Continuous-time  UseExternalTs=off  SampleTime=-1  IntegratorMethod=Forward Euler  FilterMethod=Forward Euler  ControllerParametersSource=internal  P=0.1  I=0.01  UseKiTs=off  D=0.05  UseExternalDerivativeSource=off  N=100  UseFilter=on  TunerSelectOption=Transfer Function Based (PID Tuner App)  InitialConditionSource=internal  InitialConditionForIntegrator=0  InitialConditionForFilter=0  DifferentiatorICPrevScaledInput=0  ExternalReset=none  TrackingMode=off  Kt=1  LimitOutput=off  SatLimitsSource=internal  UpperSaturationLimit=inf  LowerSaturationLimit=-inf  LinearizeAsGain=on  AntiWindupMode=none  Kb=1  LimitIntegrator=off  UpperIntegratorSaturationLimit=inf  LowerIntegratorSaturationLimit=-inf  POutMin=[]  POutMax=[]  IOutMin=[]  IOutMax=[]  DOutMin=[]  DOutMax=[]  NOutMin=[]  NOutMax=[]  SumOutMin=[]  SumOutMax=[]  SaturationOutMin=[]  SaturationOutMax=[]  PParamMin=[]  PParamMax=[]  IParamMin=[]  IParamMax=[]  DParamMin=[]  DParamMax=[]  NParamMin=[]  NParamMax=[]  KbParamMin=[]  KbParamMax=[]  KtParamMin=[]  KtParamMax=[]  KbOutMin=[]  KbOutMax=[]  KtOutMin=[]  KtOutMax=[]  IntegratorOutMin=[]  IntegratorOutMax=[]  FilterOutMin=[]  FilterOutMax=[]  SumI1OutMin=[]  SumI1OutMax=[]  SumI2OutMin=[]  SumI2OutMax=[]  SumI3OutMin=[]  SumI3OutMax=[]  SumI4OutMin=[]  SumI4OutMax=[]  SumDOutMin=[]  SumDOutMax=[]  DifferentiatorOutMin=[]  DifferentiatorOutMax=[]  FilterDiffOutCoefMin=[]  FilterDiffOutCoefMax=[]  ReciprocalOutMin=[]  ReciprocalOutMax=[]  SumDenOutMin=[]  SumDenOutMax=[]  SumNumOutMin=[]  SumNumOutMax=[]  DivideOutMin=[]  DivideOutMax=[]  UdiffTsProdOutMin=[]  UdiffTsProdOutMax=[]  NTsProdOutMin=[]  NTsProdOutMax=[]  UintegralTsProdOutMin=[]  UintegralTsProdOutMax=[]  UngainTsProdOutMin=[]  UngainTsProdOutMax=[]  ClampingZeroOutDataTypeStr=Inherit: Inherit via back propagation  ClampingZeroOutMin=[]  ClampingZeroOutMax=[]  FilterDenConstantOutDataTypeStr=Inherit: Inherit via back propagation  FilterDenConstantOutMin=[]  FilterDenConstantOutMax=[]  PCopyOutDataTypeStr=Inherit: Inherit via back propagation  PCopyOutMin=[]  PCopyOutMax=[]  NCopyOutDataTypeStr=Inherit: Inherit via back propagation  NCopyOutMin=[]  NCopyOutMax=[]  IntegratorContinuousStateAttributes=''  IntegratorStateMustResolveToSignalObject=off  IntegratorRTWStateStorageClass=Auto  FilterContinuousStateAttributes=''  FilterStateMustResolveToSignalObject=off  FilterRTWStateStorageClass=Auto  ParallelPVariant=InternalParameters  IdealPVariant=Disabled  IVariant=InternalParameters  DVariant=InternalParameters  IntegratorVariant=Continuous  SatVariant=Disabled  AWVariant=Passthrough  PCopyVariant=Disabled  TRVariant=Disabled  FdbkBlocksVariant=Forward  IdealPFdbkVariant=Disabled  SatFdbkVariant=Disabled  DerivativeFilterVariant=ContFilter  NVariant=InternalParameters  NCopyVariant=Disabled  FilterICVariant=InternalICsFilter  IntegratorICVariant=InternalICs  ExternalResetVariant=Disabled  TRSumVariant=Passthrough  SumFdbkVariant=Disabled  SumVariant=Sum_PID  TsampFilterVariant=InternalTs  TsampNgainVariant=Passthrough  TsampIntegralVariant=Disabled_SignalSpec  ExternalSaturationOutDataTypeStr=Inherit: Same as second input  DerivativeSourceVariant=ErrorSignal  PreIntVariant=InternalPreInt
  PID Controller6 : slpidlib/PID Controller  Controller=PID  Form=Parallel  TimeDomain=Continuous-time  UseExternalTs=off  SampleTime=-1  IntegratorMethod=Forward Euler  FilterMethod=Forward Euler  ControllerParametersSource=internal  P=0.1  I=0.01  UseKiTs=off  D=0.06  UseExternalDerivativeSource=off  N=100  UseFilter=on  TunerSelectOption=Transfer Function Based (PID Tuner App)  InitialConditionSource=internal  InitialConditionForIntegrator=0  InitialConditionForFilter=0  DifferentiatorICPrevScaledInput=0  ExternalReset=none  TrackingMode=off  Kt=1  LimitOutput=off  SatLimitsSource=internal  UpperSaturationLimit=inf  LowerSaturationLimit=-inf  LinearizeAsGain=on  AntiWindupMode=none  Kb=1  LimitIntegrator=off  UpperIntegratorSaturationLimit=inf  LowerIntegratorSaturationLimit=-inf  POutMin=[]  POutMax=[]  IOutMin=[]  IOutMax=[]  DOutMin=[]  DOutMax=[]  NOutMin=[]  NOutMax=[]  SumOutMin=[]  SumOutMax=[]  SaturationOutMin=[]  SaturationOutMax=[]  PParamMin=[]  PParamMax=[]  IParamMin=[]  IParamMax=[]  DParamMin=[]  DParamMax=[]  NParamMin=[]  NParamMax=[]  KbParamMin=[]  KbParamMax=[]  KtParamMin=[]  KtParamMax=[]  KbOutMin=[]  KbOutMax=[]  KtOutMin=[]  KtOutMax=[]  IntegratorOutMin=[]  IntegratorOutMax=[]  FilterOutMin=[]  FilterOutMax=[]  SumI1OutMin=[]  SumI1OutMax=[]  SumI2OutMin=[]  SumI2OutMax=[]  SumI3OutMin=[]  SumI3OutMax=[]  SumI4OutMin=[]  SumI4OutMax=[]  SumDOutMin=[]  SumDOutMax=[]  DifferentiatorOutMin=[]  DifferentiatorOutMax=[]  FilterDiffOutCoefMin=[]  FilterDiffOutCoefMax=[]  ReciprocalOutMin=[]  ReciprocalOutMax=[]  SumDenOutMin=[]  SumDenOutMax=[]  SumNumOutMin=[]  SumNumOutMax=[]  DivideOutMin=[]  DivideOutMax=[]  UdiffTsProdOutMin=[]  UdiffTsProdOutMax=[]  NTsProdOutMin=[]  NTsProdOutMax=[]  UintegralTsProdOutMin=[]  UintegralTsProdOutMax=[]  UngainTsProdOutMin=[]  UngainTsProdOutMax=[]  ClampingZeroOutDataTypeStr=Inherit: Inherit via back propagation  ClampingZeroOutMin=[]  ClampingZeroOutMax=[]  FilterDenConstantOutDataTypeStr=Inherit: Inherit via back propagation  FilterDenConstantOutMin=[]  FilterDenConstantOutMax=[]  PCopyOutDataTypeStr=Inherit: Inherit via back propagation  PCopyOutMin=[]  PCopyOutMax=[]  NCopyOutDataTypeStr=Inherit: Inherit via back propagation  NCopyOutMin=[]  NCopyOutMax=[]  IntegratorContinuousStateAttributes=''  IntegratorStateMustResolveToSignalObject=off  IntegratorRTWStateStorageClass=Auto  FilterContinuousStateAttributes=''  FilterStateMustResolveToSignalObject=off  FilterRTWStateStorageClass=Auto  ParallelPVariant=InternalParameters  IdealPVariant=Disabled  IVariant=InternalParameters  DVariant=InternalParameters  IntegratorVariant=Continuous  SatVariant=Disabled  AWVariant=Passthrough  PCopyVariant=Disabled  TRVariant=Disabled  FdbkBlocksVariant=Forward  IdealPFdbkVariant=Disabled  SatFdbkVariant=Disabled  DerivativeFilterVariant=ContFilter  NVariant=InternalParameters  NCopyVariant=Disabled  FilterICVariant=InternalICsFilter  IntegratorICVariant=InternalICs  ExternalResetVariant=Disabled  TRSumVariant=Passthrough  SumFdbkVariant=Disabled  SumVariant=Sum_PID  TsampFilterVariant=InternalTs  TsampNgainVariant=Passthrough  TsampIntegralVariant=Disabled_SignalSpec  ExternalSaturationOutDataTypeStr=Inherit: Same as second input  DerivativeSourceVariant=ErrorSignal  PreIntVariant=InternalPreInt
  PID Controller7 : slpidlib/PID Controller  Controller=PID  Form=Parallel  TimeDomain=Continuous-time  UseExternalTs=off  SampleTime=-1  IntegratorMethod=Forward Euler  FilterMethod=Forward Euler  ControllerParametersSource=internal  P=0.095  I=0.01  UseKiTs=off  D=0.07  UseExternalDerivativeSource=off  N=100  UseFilter=on  TunerSelectOption=Transfer Function Based (PID Tuner App)  InitialConditionSource=internal  InitialConditionForIntegrator=0  InitialConditionForFilter=0  DifferentiatorICPrevScaledInput=0  ExternalReset=none  TrackingMode=off  Kt=1  LimitOutput=off  SatLimitsSource=internal  UpperSaturationLimit=inf  LowerSaturationLimit=-inf  LinearizeAsGain=on  AntiWindupMode=none  Kb=1  LimitIntegrator=off  UpperIntegratorSaturationLimit=inf  LowerIntegratorSaturationLimit=-inf  POutMin=[]  POutMax=[]  IOutMin=[]  IOutMax=[]  DOutMin=[]  DOutMax=[]  NOutMin=[]  NOutMax=[]  SumOutMin=[]  SumOutMax=[]  SaturationOutMin=[]  SaturationOutMax=[]  PParamMin=[]  PParamMax=[]  IParamMin=[]  IParamMax=[]  DParamMin=[]  DParamMax=[]  NParamMin=[]  NParamMax=[]  KbParamMin=[]  KbParamMax=[]  KtParamMin=[]  KtParamMax=[]  KbOutMin=[]  KbOutMax=[]  KtOutMin=[]  KtOutMax=[]  IntegratorOutMin=[]  IntegratorOutMax=[]  FilterOutMin=[]  FilterOutMax=[]  SumI1OutMin=[]  SumI1OutMax=[]  SumI2OutMin=[]  SumI2OutMax=[]  SumI3OutMin=[]  SumI3OutMax=[]  SumI4OutMin=[]  SumI4OutMax=[]  SumDOutMin=[]  SumDOutMax=[]  DifferentiatorOutMin=[]  DifferentiatorOutMax=[]  FilterDiffOutCoefMin=[]  FilterDiffOutCoefMax=[]  ReciprocalOutMin=[]  ReciprocalOutMax=[]  SumDenOutMin=[]  SumDenOutMax=[]  SumNumOutMin=[]  SumNumOutMax=[]  DivideOutMin=[]  DivideOutMax=[]  UdiffTsProdOutMin=[]  UdiffTsProdOutMax=[]  NTsProdOutMin=[]  NTsProdOutMax=[]  UintegralTsProdOutMin=[]  UintegralTsProdOutMax=[]  UngainTsProdOutMin=[]  UngainTsProdOutMax=[]  ClampingZeroOutDataTypeStr=Inherit: Inherit via back propagation  ClampingZeroOutMin=[]  ClampingZeroOutMax=[]  FilterDenConstantOutDataTypeStr=Inherit: Inherit via back propagation  FilterDenConstantOutMin=[]  FilterDenConstantOutMax=[]  PCopyOutDataTypeStr=Inherit: Inherit via back propagation  PCopyOutMin=[]  PCopyOutMax=[]  NCopyOutDataTypeStr=Inherit: Inherit via back propagation  NCopyOutMin=[]  NCopyOutMax=[]  IntegratorContinuousStateAttributes=''  IntegratorStateMustResolveToSignalObject=off  IntegratorRTWStateStorageClass=Auto  FilterContinuousStateAttributes=''  FilterStateMustResolveToSignalObject=off  FilterRTWStateStorageClass=Auto  ParallelPVariant=InternalParameters  IdealPVariant=Disabled  IVariant=InternalParameters  DVariant=InternalParameters  IntegratorVariant=Continuous  SatVariant=Disabled  AWVariant=Passthrough  PCopyVariant=Disabled  TRVariant=Disabled  FdbkBlocksVariant=Forward  IdealPFdbkVariant=Disabled  SatFdbkVariant=Disabled  DerivativeFilterVariant=ContFilter  NVariant=InternalParameters  NCopyVariant=Disabled  FilterICVariant=InternalICsFilter  IntegratorICVariant=InternalICs  ExternalResetVariant=Disabled  TRSumVariant=Passthrough  SumFdbkVariant=Disabled  SumVariant=Sum_PID  TsampFilterVariant=InternalTs  TsampNgainVariant=Passthrough  TsampIntegralVariant=Disabled_SignalSpec  ExternalSaturationOutDataTypeStr=Inherit: Same as second input  DerivativeSourceVariant=ErrorSignal  PreIntVariant=InternalPreInt
  PID Working : slpidlib/PID Controller  Controller=PI  Form=Parallel  TimeDomain=Continuous-time  UseExternalTs=off  SampleTime=-1  IntegratorMethod=Forward Euler  FilterMethod=Forward Euler  ControllerParametersSource=internal  P=0.1  I=0.01  UseKiTs=off  D=0  UseExternalDerivativeSource=off  N=100  UseFilter=on  TunerSelectOption=Transfer Function Based (PID Tuner App)  InitialConditionSource=internal  InitialConditionForIntegrator=0  InitialConditionForFilter=0  DifferentiatorICPrevScaledInput=0  ExternalReset=none  TrackingMode=off  Kt=1  LimitOutput=off  SatLimitsSource=internal  UpperSaturationLimit=inf  LowerSaturationLimit=-inf  LinearizeAsGain=on  AntiWindupMode=none  Kb=1  LimitIntegrator=off  UpperIntegratorSaturationLimit=inf  LowerIntegratorSaturationLimit=-inf  POutMin=[]  POutMax=[]  IOutMin=[]  IOutMax=[]  DOutMin=[]  DOutMax=[]  NOutMin=[]  NOutMax=[]  SumOutMin=[]  SumOutMax=[]  SaturationOutMin=[]  SaturationOutMax=[]  PParamMin=[]  PParamMax=[]  IParamMin=[]  IParamMax=[]  DParamMin=[]  DParamMax=[]  NParamMin=[]  NParamMax=[]  KbParamMin=[]  KbParamMax=[]  KtParamMin=[]  KtParamMax=[]  KbOutMin=[]  KbOutMax=[]  KtOutMin=[]  KtOutMax=[]  IntegratorOutMin=[]  IntegratorOutMax=[]  FilterOutMin=[]  FilterOutMax=[]  SumI1OutMin=[]  SumI1OutMax=[]  SumI2OutMin=[]  SumI2OutMax=[]  SumI3OutMin=[]  SumI3OutMax=[]  SumI4OutMin=[]  SumI4OutMax=[]  SumDOutMin=[]  SumDOutMax=[]  DifferentiatorOutMin=[]  DifferentiatorOutMax=[]  FilterDiffOutCoefMin=[]  FilterDiffOutCoefMax=[]  ReciprocalOutMin=[]  ReciprocalOutMax=[]  SumDenOutMin=[]  SumDenOutMax=[]  SumNumOutMin=[]  SumNumOutMax=[]  DivideOutMin=[]  DivideOutMax=[]  UdiffTsProdOutMin=[]  UdiffTsProdOutMax=[]  NTsProdOutMin=[]  NTsProdOutMax=[]  UintegralTsProdOutMin=[]  UintegralTsProdOutMax=[]  UngainTsProdOutMin=[]  UngainTsProdOutMax=[]  ClampingZeroOutDataTypeStr=Inherit: Inherit via back propagation  ClampingZeroOutMin=[]  ClampingZeroOutMax=[]  FilterDenConstantOutDataTypeStr=Inherit: Inherit via back propagation  FilterDenConstantOutMin=[]  FilterDenConstantOutMax=[]  PCopyOutDataTypeStr=Inherit: Inherit via back propagation  PCopyOutMin=[]  PCopyOutMax=[]  NCopyOutDataTypeStr=Inherit: Inherit via back propagation  NCopyOutMin=[]  NCopyOutMax=[]  IntegratorContinuousStateAttributes=''  IntegratorStateMustResolveToSignalObject=off  IntegratorRTWStateStorageClass=Auto  FilterContinuousStateAttributes=''  FilterStateMustResolveToSignalObject=off  FilterRTWStateStorageClass=Auto  ParallelPVariant=InternalParameters  IdealPVariant=Disabled  IVariant=InternalParameters  DVariant=Disabled  IntegratorVariant=Continuous  SatVariant=Disabled  AWVariant=Passthrough  PCopyVariant=Disabled  TRVariant=Disabled  FdbkBlocksVariant=Forward  IdealPFdbkVariant=Disabled  SatFdbkVariant=Disabled  DerivativeFilterVariant=Disabled  NVariant=Disabled  NCopyVariant=Disabled_SignalSpec  FilterICVariant=Disabled  IntegratorICVariant=InternalICs  ExternalResetVariant=Disabled  TRSumVariant=Passthrough  SumFdbkVariant=Disabled  SumVariant=Sum_PI  TsampFilterVariant=InternalTs  TsampNgainVariant=Passthrough  TsampIntegralVariant=Disabled_SignalSpec  ExternalSaturationOutDataTypeStr=Inherit: Same as second input  DerivativeSourceVariant=Disabled  PreIntVariant=InternalPreInt
  Rate Limiter5 : RateLimiter  RisingSlewLimit=3  FallingSlewLimit=-3  InitialCondition=20
  Saturation2 : Saturate  UpperLimit=15*(pi/180)  LowerLimit=-15*(pi/180)
  Scope{,1..2,4..5} (5 alike) : Scope
      Scope settings: ActiveDisplayYMinimum=2.0000000000000004  ActiveDisplayYMaximum=22  DataLoggingVariableName=ScopeData93
      Scope1 settings: ActiveDisplayYMinimum=-1  ActiveDisplayYMaximum=1  DataLoggingVariableName=ScopeData68
      Scope2 settings: ActiveDisplayYMinimum=-0.31651876722314576  ActiveDisplayYMaximum=0.50167948601670753  DataLoggingVariableName=ScopeData94
      Scope4 settings: ActiveDisplayYMinimum=2.0000000000000004  ActiveDisplayYMaximum=22  DataLoggingVariableName=ScopeData27
      Scope5 settings: ActiveDisplayYMinimum=-2.300715089643941  ActiveDisplayYMaximum=2.3531021232923295  DataLoggingVariableName=ScopeData41
  Scope3 : Scope  NumInputPorts=2
      settings: ActiveDisplayYMinimum=0.25093822790107057  ActiveDisplayYMaximum=21.821789611249248  DataLoggingVariableName=ScopeData26
  Selector1 : Selector  InputPortWidth=3  IndexOptions=Index vector (dialog)  Indices=[3]  OutputSizes=1
  Subtract1 : Sum  Inputs=+-
  Desired Pitch Angle : Outport
  wires:
  Gain4/1 -> Subtract1/2, Scope3/1  "Measured Altitude"
  Selector1/1 -> Gain4/1
  Constant5/1 -> Add3/2
  <Xe>/1 -> Selector1/1
  altitudeCmd_m/1 -> Gain5/1
  Gain5/1 -> Rate Limiter5/1, Scope4/1  "Altitude Command"
  Add3/1 -> Saturation2/1, Scope2/1
  Subtract1/1 -> PID Controller1/1, Scope5/1  "Measured Altitude"
  PID Controller1/1 -> Add3/1
  Saturation2/1 -> Desired Pitch Angle/1, Scope1/1
  Rate Limiter5/1 -> Scope/1, Scope3/2, Subtract1/1  "Commanded Altitude"

== system SIXDOF28/Subsystem2/Cross Track Controller ==
  In1 : Inport
  In2 : Inport  Port=2
  Add : Sum
  Atan2 : Trigonometry  Operator=atan2
  Constant : Constant  Value=g
  Kd : Gain  Gain=1.7
  Kp : Gain
  Saturation : Saturate  UpperLimit=30*pi/180  LowerLimit=-30*pi/180
  Scope9 : Scope
      settings: ActiveDisplayYMinimum=-1  ActiveDisplayYMaximum=1  DataLoggingVariableName=ScopeData104
  Out1 : Outport
  wires:
  Saturation/1 -> Out1/1
  Add/1 -> Scope9/1, Atan2/1
  Kp/1 -> Add/1
  Constant/1 -> Atan2/2
  Kd/1 -> Add/2
  Atan2/1 -> Saturation/1
  In2/1 -> Kd/1
  In1/1 -> Kp/1

== system SIXDOF28/Subsystem2/Flight Controller ==
  <Xe> : Inport
  waypointsNED : Inport  Port=2
  <Ve> : Inport  Port=3
  Constant4 : Constant  Value=20
  MATLAB Function1 : MATLAB Function  TreatAsAtomicUnit=on
  Scope{,2..6,8} (7 alike) : Scope
      Scope settings: DataLoggingVariableName=ScopeData51
      Scope2 settings: ActiveDisplayYMinimum=-22.562051057641373  ActiveDisplayYMaximum=15.463086611993543  DataLoggingVariableName=ScopeData98
      Scope3 settings: ActiveDisplayYMinimum=-1  ActiveDisplayYMaximum=1  DataLoggingVariableName=ScopeData99
      Scope4 settings: ActiveDisplayYMinimum=-1  ActiveDisplayYMaximum=1  DataLoggingVariableName=ScopeData100
      Scope5 settings: ActiveDisplayYMinimum=-1  ActiveDisplayYMaximum=1  DataLoggingVariableName=ScopeData101
      Scope6 settings: ActiveDisplayYMinimum=-1  ActiveDisplayYMaximum=1  DataLoggingVariableName=ScopeData102
      Scope8 settings: ActiveDisplayYMinimum=11.572741226614  ActiveDisplayYMaximum=106.6245134440201  DataLoggingVariableName=ScopeData103
  Scope1 : Scope  NumInputPorts=2
      settings: ActiveDisplayYMinimum=-22.562051057641373  ActiveDisplayYMaximum=15.463086611993543  DataLoggingVariableName=ScopeData69
  Unit Delay : UnitDelay  SampleTime=-1  HasFrameUpgradeWarning=on
  crossTrackError_m : Outport
  crossTrackRate_mps : Outport  Port=2
  altitudeCmd_m : Outport  Port=3
  wires:
  waypointsNED/1 -> MATLAB Function1/3(waypointsNED)
  MATLAB Function1/2(crossTrackRate_mps) -> Scope1/2, crossTrackRate_mps/1, Scope3/1
  Constant4/1 -> MATLAB Function1/5(waypointRadius_m)
  MATLAB Function1/4(activeLegIdxOut) -> Unit Delay/1, Scope5/1
  Unit Delay/1 -> MATLAB Function1/4(activeLegIdxIn)
  MATLAB Function1/1(crossTrackError_m) -> Scope1/1, crossTrackError_m/1, Scope2/1  "CrossTrackError"
  MATLAB Function1/8(altitudeCmd_m) -> altitudeCmd_m/1
  MATLAB Function1/6(distanceToWaypointB_m) -> Scope8/1
  MATLAB Function1/5(switchFlag) -> Scope6/1
  MATLAB Function1/3(alongTrackRate_mps) -> Scope4/1
  <Xe>/1 -> MATLAB Function1/1(vehiclePosNED)
  <Ve>/1 -> MATLAB Function1/2(vehicleVelNED)
  MATLAB Function1/7(closestPointNED) -> Scope/1
